simulink model "Safety_Chain"  (R2026b)
settings: Solver=VariableStepAuto
undefined symbols (not defined in the file or in its folder): Ts
libraries: eeGeneralControl x4, simulink x1
settings Model: Creator=aomar  LastModifiedBy=aomar

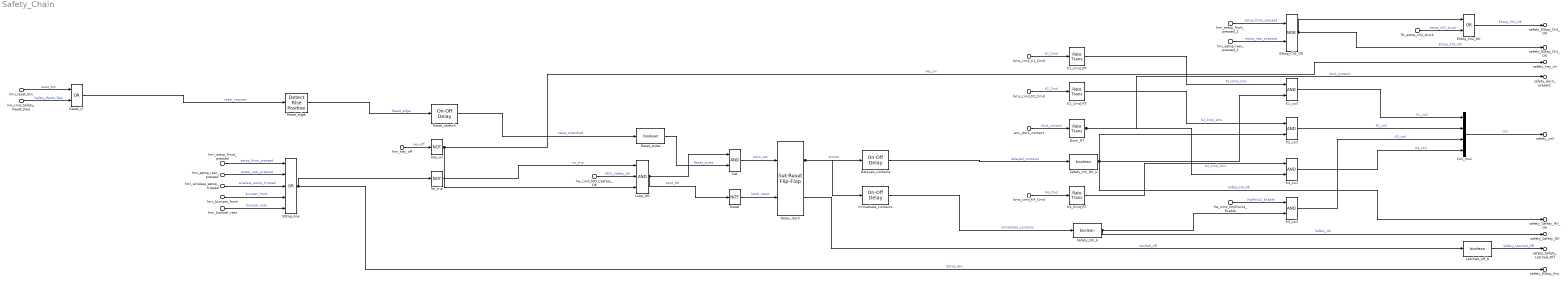
== system Safety_Chain ==
  hmi_estop_front_pressed : Inport  PortName=hmi  Element=estop_front_pressed
  hmi_estop_front_pressed_2 : Inport  PortName=hmi  Element=estop_front_pressed
  hmi_estop_rear_pressed : Inport  PortName=hmi  Element=estop_rear_pressed
  hmi_estop_rear_pressed_2 : Inport  PortName=hmi  Element=estop_rear_pressed
  hmi_wireless_estop_tripped : Inport  PortName=hmi  Element=wireless_estop_tripped
  hmi_bumper_front : Inport  PortName=hmi  Element=bumper_front
  hmi_bumper_rear : Inport  PortName=hmi  Element=bumper_rear
  hmi_key_off : Inport  PortName=hmi  Element=key_off
  hmi_reset_btn : Inport  PortName=hmi  Element=reset_btn
  hw_cmd_MCU_Safety_OK : Inport  Port=2  PortName=hw_cmd  Element=MCU_Safety_OK
  hw_cmd_Safety_Reset_Req : Inport  Port=2  PortName=hw_cmd  Element=Safety_Reset_Req
  hw_cmd_ImpPwr24_Enable : Inport  Port=2  PortName=hw_cmd  Element=ImpPwr24_Enable
  bms_cmd_K1_Cmd : Inport  Port=3  PortName=bms_cmd  Element=K1_Cmd
  bms_cmd_K2_Cmd : Inport  Port=3  PortName=bms_cmd  Element=K2_Cmd
  bms_cmd_K4_Cmd : Inport  Port=3  PortName=bms_cmd  Element=K4_Cmd
  env_dock_contact : Inport  Port=4  PortName=env  Element=dock_contact
  flt_estop_ch2_stuck : Inport  Port=5  PortName=flt  Element=estop_ch2_stuck
  Coil_mux : Mux
  Delayed_contacts : eeGeneralControl/On-Off Delay  LabelModeActiveChoice=Discrete  Td_on=P.power.safety.t_relay_on  Td_off=P.power.safety.t_cat1  IC=P.power.safety.Q0  Ts=Ts.safety
      settings: LibrarySourceBlock=ee_sl_lib/General Control/On-Off Delay
  Dock_RT : RateTransition  OutPortSampleTime=Ts.safety
  EStop_Any : Logic  Operator=OR  Inputs=5  AllPortsSameDT=off  OutDataTypeStr=boolean
  EStop_Ch1_OK : Logic  Operator=NOR  AllPortsSameDT=off  OutDataTypeStr=boolean
  EStop_Ch2_OK : Logic  Operator=OR  AllPortsSameDT=off  OutDataTypeStr=boolean
  Immediate_contacts : eeGeneralControl/On-Off Delay  LabelModeActiveChoice=Discrete  Td_on=P.power.safety.t_relay_on  Td_off=P.power.safety.t_relay_off  IC=P.power.safety.Q0  Ts=Ts.safety
      settings: LibrarySourceBlock=ee_sl_lib/General Control/On-Off Delay
  K1_Cmd_RT : RateTransition  OutPortSampleTime=Ts.safety
  K1_coil : Logic  AllPortsSameDT=off  OutDataTypeStr=boolean
  K2_Cmd_RT : RateTransition  OutPortSampleTime=Ts.safety
  K2_coil : Logic  AllPortsSameDT=off  OutDataTypeStr=boolean
  K3_coil : Logic  AllPortsSameDT=off  OutDataTypeStr=boolean
  K4_Cmd_RT : RateTransition  OutPortSampleTime=Ts.safety
  K4_coil : Logic  AllPortsSameDT=off  OutDataTypeStr=boolean
  Key_on : Logic  Operator=NOT  AllPortsSameDT=off  OutDataTypeStr=boolean
  Latched_off_b : DataTypeConversion  OutDataTypeStr=boolean  RndMeth=Nearest
  Loop_OK : Logic  Inputs=3  AllPortsSameDT=off  OutDataTypeStr=boolean
  No_trip : Logic  Operator=NOT  AllPortsSameDT=off  OutDataTypeStr=boolean
  Relay_latch : eeGeneralControl/Set-Reset Flip-Flop  LabelModeActiveChoice=Discrete  UndefState=Reset  Q0=P.power.safety.Q0  Ts=Ts.safety
      settings: LibrarySourceBlock=ee_sl_lib/General Control/Set-Reset Flip-Flop
  Reset : Logic  Operator=NOT  AllPortsSameDT=off  OutDataTypeStr=boolean
  Reset_edge : simulink/Logic and Bit Operations/Detect Rise Positive  vinit=0  OutDataTypeStr=boolean
  Reset_in : Logic  Operator=OR  AllPortsSameDT=off  OutDataTypeStr=boolean
  Reset_pulse : DataTypeConversion  OutDataTypeStr=boolean  RndMeth=Nearest
  Reset_stretch : eeGeneralControl/On-Off Delay  LabelModeActiveChoice=Discrete  Td_on=0  Td_off=P.power.safety.t_reset_hold  IC=0  Ts=Ts.safety
      settings: LibrarySourceBlock=ee_sl_lib/General Control/On-Off Delay
  Safety_HV_OK_b : DataTypeConversion  OutDataTypeStr=boolean  RndMeth=Nearest
  Safety_OK_b : DataTypeConversion  OutDataTypeStr=boolean  RndMeth=Nearest
  Set : Logic  AllPortsSameDT=off  OutDataTypeStr=boolean
  safety_Safety_OK : Outport  PortName=safety  Element=Safety_OK
  safety_Safety_HV_OK : Outport  PortName=safety  Element=Safety_HV_OK
  safety_EStop_Any : Outport  PortName=safety  Element=EStop_Any
  safety_EStop_Ch1_OK : Outport  PortName=safety  Element=EStop_Ch1_OK
  safety_EStop_Ch2_OK : Outport  PortName=safety  Element=EStop_Ch2_OK
  safety_Safety_Latched_Off : Outport  PortName=safety  Element=Safety_Latched_Off
  safety_coil : Outport  PortName=safety  Element=coil
  safety_key_on : Outport  PortName=safety  Element=key_on
  safety_dock_present : Outport  PortName=safety  Element=dock_present
  wires:
  hmi_reset_btn/1 -> Reset_in/1  "reset_btn"
  hw_cmd_Safety_Reset_Req/1 -> Reset_in/2  "Safety_Reset_Req"
  Reset_in/1 -> Reset_edge/1  "reset_request"
  hmi_estop_front_pressed/1 -> EStop_Any/1  "estop_front_pressed"
  hmi_estop_rear_pressed/1 -> EStop_Any/2  "estop_rear_pressed"
  hmi_wireless_estop_tripped/1 -> EStop_Any/3  "wireless_estop_tripped"
  hmi_bumper_front/1 -> EStop_Any/4  "bumper_front"
  hmi_bumper_rear/1 -> EStop_Any/5  "bumper_rear"
  EStop_Any/1 -> safety_EStop_Any/1, No_trip/1  "EStop_Any"
  Reset_edge/1 -> Reset_stretch/1  "Reset_edge"
  hmi_key_off/1 -> Key_on/1  "key_off"
  Key_on/1 -> safety_key_on/1, Loop_OK/3  "key_on"
  No_trip/1 -> Loop_OK/1  "no_trip"
  Reset_stretch/1 -> Reset_pulse/1  "reset_stretched"
  hw_cmd_MCU_Safety_OK/1 -> Loop_OK/2  "MCU_Safety_OK"
  Loop_OK/1 -> Set/1, Reset/1  "Loop_OK"
  Reset_pulse/1 -> Set/2  "Reset_pulse"
  Set/1 -> Relay_latch/1  "latch_set"
  Reset/1 -> Relay_latch/2  "latch_reset"
  Relay_latch/1 -> Immediate_contacts/1, Delayed_contacts/1  "Armed"
  Relay_latch/2 -> Latched_off_b/1  "latched_off"
  Delayed_contacts/1 -> Safety_HV_OK_b/1  "delayed_contacts"
  Immediate_contacts/1 -> Safety_OK_b/1  "immediate_contacts"
  bms_cmd_K1_Cmd/1 -> K1_Cmd_RT/1  "K1_Cmd"
  bms_cmd_K2_Cmd/1 -> K2_Cmd_RT/1  "K2_Cmd"
  env_dock_contact/1 -> Dock_RT/1  "dock_contact"
  bms_cmd_K4_Cmd/1 -> K4_Cmd_RT/1  "K4_Cmd"
  K1_Cmd_RT/1 -> K1_coil/1  "K1_Cmd_1ms"
  K2_Cmd_RT/1 -> K2_coil/1  "K2_Cmd_1ms"
  Dock_RT/1 -> safety_dock_present/1, K4_coil/2  "dock_present"
  K4_Cmd_RT/1 -> K4_coil/1  "K4_Cmd_1ms"
  Safety_HV_OK_b/1 -> K1_coil/2, safety_Safety_HV_OK/1, K2_coil/2  "Safety_HV_OK"
  Safety_OK_b/1 -> K3_coil/2, safety_Safety_OK/1  "Safety_OK"
  hmi_estop_front_pressed_2/1 -> EStop_Ch1_OK/1  "estop_front_pressed"
  hmi_estop_rear_pressed_2/1 -> EStop_Ch1_OK/2  "estop_rear_pressed"
  hw_cmd_ImpPwr24_Enable/1 -> K3_coil/1  "ImpPwr24_Enable"
  EStop_Ch1_OK/1 -> safety_EStop_Ch1_OK/1, EStop_Ch2_OK/1  "EStop_Ch1_OK"
  K1_coil/1 -> Coil_mux/1  "K1_coil"
  K2_coil/1 -> Coil_mux/2  "K2_coil"
  K4_coil/1 -> Coil_mux/4  "K4_coil"
  K3_coil/1 -> Coil_mux/3  "K3_coil"
  flt_estop_ch2_stuck/1 -> EStop_Ch2_OK/2  "estop_ch2_stuck"
  Coil_mux/1 -> safety_coil/1  "coil"
  EStop_Ch2_OK/1 -> safety_EStop_Ch2_OK/1  "EStop_Ch2_OK"
  Latched_off_b/1 -> safety_Safety_Latched_Off/1  "Safety_Latched_Off"
